simulink model "dc_motor_statespace"  (R2026a)
settings: Solver=ode45  StopTime=30  MaxStep=0.001  RelTol=1e-08  AbsTol=1e-10
model workspace (MAT data in the model file):
  A = [-4  -0.2; 3.33333333333  -0.0333333333333]
  B = [2  0; 0  -33.3333333333]
  C = [0  1; 1  0]
  D = [0  0; 0  0]
  TorqueTime = 1
  TorqueValue = 0
  VinValue = 12
  p.Ra = 2
  p.La = 0.5
  p.Kt = 0.1
  p.Ke = 0.1
  p.Jm = 0.01
  p.Bm = 0.001
  p.JL = 0.02
  p.J = 0.03
  p.B = 0.001
  p.w_ref = 100
  p.Vmin = -48
  p.Vmax = 48
  p.beta = 1
  p.gamma = 0
  p.derivativeRatio = 20
  p.minimumFilterTime = 0.001
  p.ts_spec = 2
  p.os_spec = 5
  p.ess_spec = 0.2
  p.band = 0.02
  p.dt = 0.001
  p.RelTol = 1e-08
  p.AbsTol = 1e-10
  p.seed = 7
  p.Tsim = 5
  p.Tsim_ol = 30
  p.TL_step = 0.05
  p.TL_time = 1
  p.config.schemaVersion = 1
  p.config.physical.Ra = 2
  p.config.physical.La = 0.5
  p.config.physical.Kt = 0.1
  p.config.physical.Ke = 0.1
  p.config.physical.Jm = 0.01
  p.config.physical.Bm = 0.001
  p.config.physical.JL = 0.02
  p.config.control.reference = 100
  p.config.control.Vmin = -48
  p.config.control.Vmax = 48
  p.config.control.beta = 1
  p.config.control.gamma = 0
  p.config.control.derivativeRatio = 20
  p.config.control.minimumFilterTime = 0.001
  p.config.control.antiWindup = 'back-calculation'
  p.config.chosenTargets.settlingBand = 0.02
  p.config.chosenTargets.settlingTime = 2
  p.config.chosenTargets.overshootPercent = 5
  p.config.chosenTargets.steadyError = 0.2
  p.config.numerics.relativeTolerance = 1e-08
  p.config.numerics.absoluteTolerance = 1e-10
  p.config.numerics.outputStep = 0.001
  p.config.numerics.seed = 7
  p.config.assumptions = {'Bipolar +/-48 V is an engineering choice; the assignment specifies no voltage limit.'; 'Overshoot <=5% and steady error <=0.2 rad/s are chosen targets, not instructor-specified limits.'; 'The rigid load adds inertia only. Positive load torque opposes positive rotation.'}
  x0 = [0; 0]
settings Model: Creator=ievge  LastModifiedBy=ievge

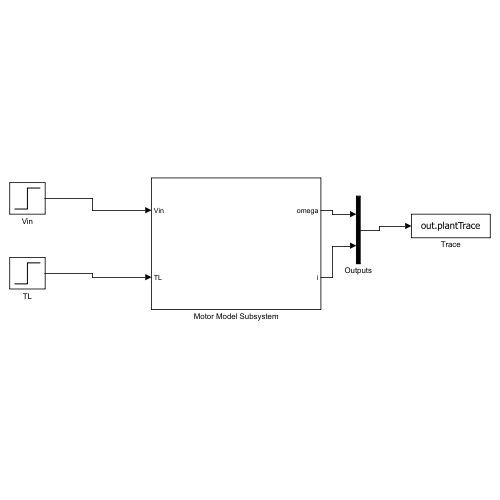
[thumbnail: Simulink's stored preview of the top-level diagram]
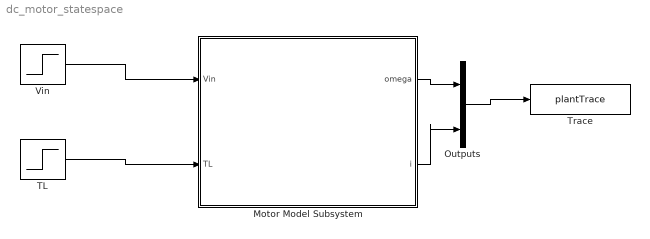
== system dc_motor_statespace ==
  Motor Model Subsystem : Subsystem
  Outputs : Mux  Inputs=2
  TL : Step  Time=TorqueTime  FinalValue=TorqueValue  SampleTime=0
  Trace : ToWorkspace  VariableName=plantTrace  SaveFormat=Timeseries  SampleTime=-1
  Vin : Step  Time=0  FinalValue=VinValue  SampleTime=0
  wires:
  Vin/1 -> Motor Model Subsystem/1(Vin)
  TL/1 -> Motor Model Subsystem/2(TL)
  Motor Model Subsystem/1(omega) -> Outputs/1
  Motor Model Subsystem/2(i) -> Outputs/2
  Outputs/1 -> Trace/1

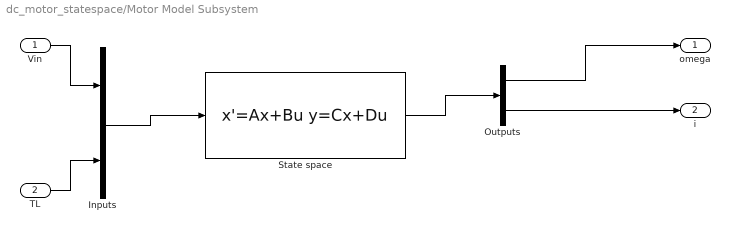
== system dc_motor_statespace/Motor Model Subsystem ==
  Vin : Inport
  TL : Inport  Port=2
  Inputs : Mux  Inputs=2
  Outputs : Demux  Outputs=2
  State space : StateSpace  A=A  B=B  C=C  D=D  InitialCondition=x0
  omega : Outport
  i : Outport  Port=2
  wires:
  Vin/1 -> Inputs/1
  TL/1 -> Inputs/2
  Inputs/1 -> State space/1
  State space/1 -> Outputs/1
  Outputs/1 -> omega/1
  Outputs/2 -> i/1
